simulink model "ASEComTestB"  (R2025a)
settings: Solver=ode4  StartTime=0.0  StopTime=inf  FixedStep=0.01  RelTol=1e-3
libraries: simulink x13, ASEToolBox x4
settings Model: Creator=admin  LastModifiedBy=zqhkd
settings DataIOCC: SaveFinalState=on  SaveOutput=off  InspectSignalLogs=on  SaveTime=off
settings OptimizationCC: EnhancedBackFolding=on  PassReuseOutputArgsAs=Individual arguments  ZeroExternalMemoryAtStartup=off  ZeroInternalMemoryAtStartup=off  OptimizeBlockOrder=speed  DifferentSizesBufferReuse=on  OptimizationCustomize=off  EfficientTunableParamExpr=on
settings DebuggingCC: ParameterTunabilityLossMsg=error
settings HardwareCC: ProdBitPerLong=64.0  ProdHWDeviceType=Intel->x86-64 (Linux 64)
settings SFSimCC: MATLABDynamicMemAlloc=off
settings RTWCC: SystemTargetFile=ert.tlc  TemplateMakefile=ert_default_tmf  RetainRTWFile=on  Toolchain=LCC-win64 v2.4.1 | gmake (64-bit Windows)  GPUComputeCapability=3.5  Description=Embedded Coder
settings CodeAppCC: ForceParamTrailComments=on  IgnoreCustomStorageClasses=off  OperatorAnnotations=on  SimulinkDataObjDesc=on  SFDataObjDesc=on  InsertBlockDesc=on
settings ERTTargetCC: ExtModeTransport=0.0  ExtModeStaticAlloc=off  ExtModeMexFile=ext_comm  ExtModeIntrfLevel=Level1  InlinedParameterPlacement=Hierarchical  RTWCAPISignals=on  RTWCAPIParams=on  RTWCAPIStates=on  RTWCAPIRootIO=on  ERTCustomFileTemplate=example_file_process.tlc  DynamicArrayContainerType=coder::array  TargetLangStandard=C99 (ISO)  SupportContinuousTime=on

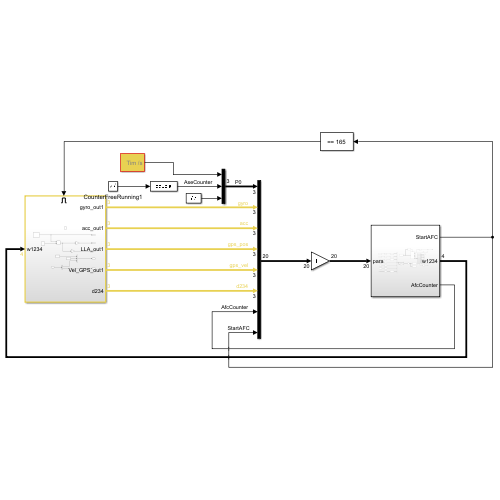
[thumbnail: Simulink's stored preview of the top-level diagram]
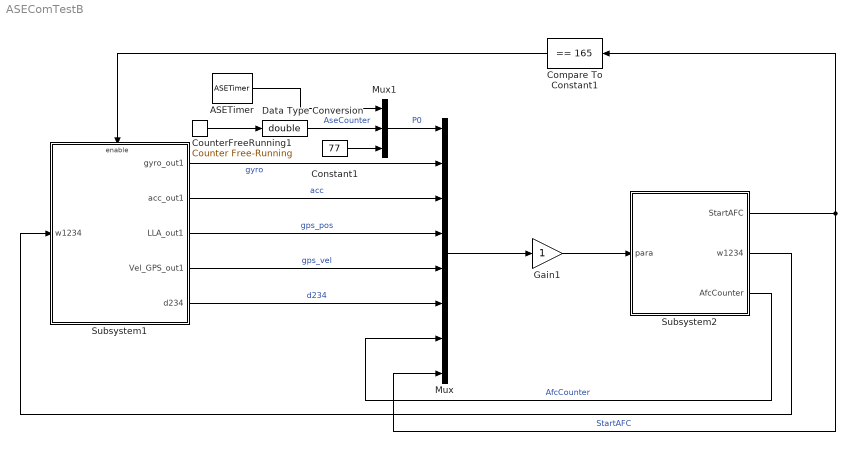
== system ASEComTestB ==
  ASETimer : ASEToolBox/SIMSystemModule/ASETimer  Priority=0  g_sampleTime=0.02
      settings: SourceProductName=ASEToolBox
  Compare To Constant1 : simulink/Logic and Bit Operations/Compare To Constant  relop===  const=165  OutDataTypeStr=boolean
  Constant1 : Constant  Value=77
  CounterFreeRunning1 : simulink/Sources/Counter Free-Running  NumBits=32  tsamp=-1
  Data Type Conversion : DataTypeConversion  OutDataTypeStr=double  SaturateOnIntegerOverflow=off  RndMeth=Floor
  Gain1 : Gain
  Mux : Mux  Inputs=8
  Mux1 : Mux  Inputs=3
  Subsystem1 : Subsystem
  Subsystem2 : Subsystem  Priority=5
  wires:
  Mux/1 -> Gain1/1
  Subsystem2/1(StartAFC) -> Mux/8, Compare To Constant1/1  "StartAFC"
  Gain1/1 -> Subsystem2/1(para)
  Compare To Constant1/1 -> Subsystem1/Enable
  Subsystem1/1(gyro_out1) -> Mux/2  "gyro"
  Subsystem1/2(acc_out1) -> Mux/3  "acc"
  Subsystem1/4(Vel_GPS_out1) -> Mux/5  "gps_vel"
  Subsystem1/5(d234) -> Mux/6  "d234"
  Subsystem2/3(AfcCounter) -> Mux/7  "AfcCounter"
  Subsystem2/2(w1234) -> Subsystem1/1(w1234)
  CounterFreeRunning1/1 -> Data Type Conversion/1
  Mux1/1 -> Mux/1  "P0"
  Subsystem1/3(LLA_out1) -> Mux/4  "gps_pos"
  ASETimer/1 -> Mux1/1
  Data Type Conversion/1 -> Mux1/2  "AseCounter"
  Constant1/1 -> Mux1/3

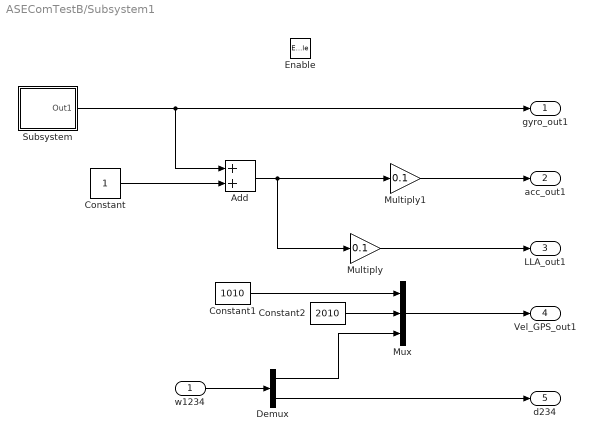
== system ASEComTestB/Subsystem1 ==
  w1234 : Inport
  Enable : EnablePort
  Add : Sum
  Constant : Constant
  Constant1 : Constant  Value=1010
  Constant2 : Constant  Value=2010
  Demux : Demux  Outputs=[1,3]
  Multiply : Gain  Gain=0.1
  Multiply1 : Gain  Gain=0.1
  Mux : Mux  Inputs=3
  Subsystem : Subsystem
  gyro_out1 : Outport
  acc_out1 : Outport  Port=2
  LLA_out1 : Outport  Port=3
  Vel_GPS_out1 : Outport  Port=4
  d234 : Outport  Port=5
  wires:
  w1234/1 -> Demux/1
  Subsystem/1(Out1) -> Add/1, gyro_out1/1
  Add/1 -> Multiply/1, Multiply1/1
  Constant/1 -> Add/2
  Multiply/1 -> LLA_out1/1
  Constant1/1 -> Mux/1
  Demux/1 -> Mux/3
  Mux/1 -> Vel_GPS_out1/1
  Demux/2 -> d234/1
  Multiply1/1 -> acc_out1/1
  Constant2/1 -> Mux/2

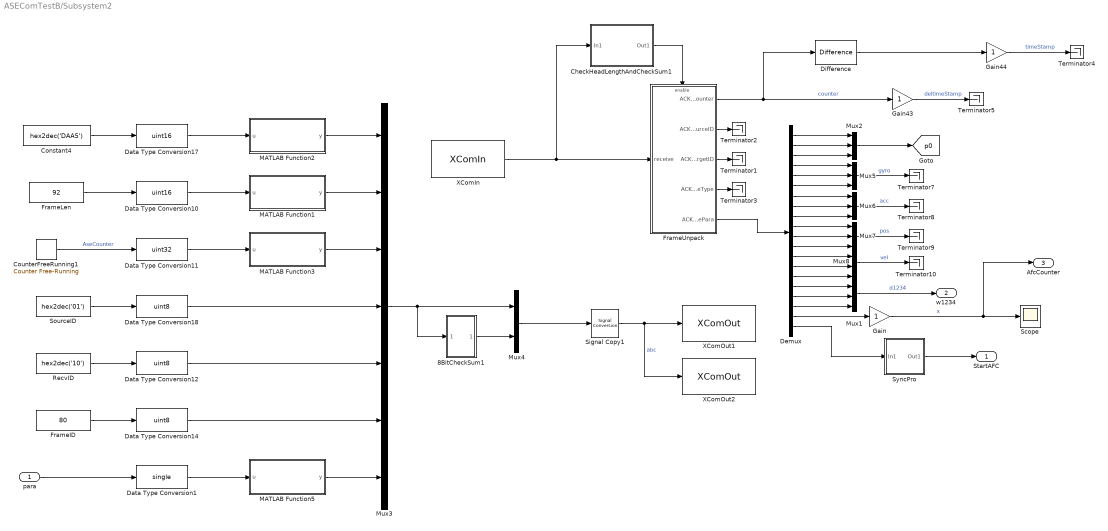
== system ASEComTestB/Subsystem2 ==
  para : Inport  PortDimensions=20
  8BitCheckSum1 : Subsystem
  CheckHeadLengthAndCheckSum1 : Subsystem
  Constant4 : Constant  Value=hex2dec('DAA5')
  CounterFreeRunning1 : simulink/Sources/Counter Free-Running  NumBits=32  tsamp=-1
  Data Type Conversion1 : DataTypeConversion  OutDataTypeStr=single  SaturateOnIntegerOverflow=off  RndMeth=Floor
  Data Type Conversion10 : DataTypeConversion  OutDataTypeStr=uint16  SaturateOnIntegerOverflow=off  RndMeth=Floor
  Data Type Conversion11 : DataTypeConversion  OutDataTypeStr=uint32  SaturateOnIntegerOverflow=off  RndMeth=Floor
  Data Type Conversion12 : DataTypeConversion  OutDataTypeStr=uint8  SaturateOnIntegerOverflow=off  RndMeth=Floor
  Data Type Conversion14 : DataTypeConversion  OutDataTypeStr=uint8  SaturateOnIntegerOverflow=off  RndMeth=Floor
  Data Type Conversion17 : DataTypeConversion  OutDataTypeStr=uint16  SaturateOnIntegerOverflow=off  RndMeth=Floor
  Data Type Conversion18 : DataTypeConversion  OutDataTypeStr=uint8  SaturateOnIntegerOverflow=off  RndMeth=Floor
  Demux : Demux  Outputs=20
  Difference : simulink/Discrete/Difference  ICPrevInput=0.0  OutMin=[]  OutMax=[]  OutDataType=fixdt(1, 16)  OutScaling=2^-10  DoSatur=off
  FrameID : Constant  Value=80
  FrameLen : Constant  Value=92
  FrameUnpack : Subsystem
  Gain : Gain
  Gain43 : Gain  OutDataTypeStr=Inherit: Same as input
  Gain44 : Gain  OutDataTypeStr=Inherit: Same as input
  MATLAB Function1 : MATLAB Function  TreatAsAtomicUnit=on
  MATLAB Function2 : MATLAB Function  TreatAsAtomicUnit=on
  MATLAB Function3 : MATLAB Function  TreatAsAtomicUnit=on
  MATLAB Function5 : MATLAB Function  TreatAsAtomicUnit=on
  Mux1 : Mux
  Mux{2,5..7} (4 alike) : Mux  Inputs=3
  Mux3 : Mux  Inputs=7
  Mux4 : Mux  Inputs=2
  Mux8 : Mux  Inputs=2
  RecvID : Constant  Value=hex2dec('10')
  Scope : Scope
  Signal Copy1 : SignalConversion  OverrideOpt=on
  SourceID : Constant  Value=hex2dec('01')
  SyncPro : Subsystem
  Terminator{1..5,7..10} (9 alike) : Terminator
  XComIn : ASEToolBox/COMModule/XComIn  g_serial_select=ttyS1  g_baudrate=460800  g_parity=None  g_databit=8  g_stopbit=0  g_data_size=92  g_sample_time=-1
      settings: SourceProductName=ASEToolBox
  XComOut1 : ASEToolBox/COMModule/XComOut  g_serial_select=ttyS1  g_baudrate=460800  g_parity=None  g_databit=8  g_stopbit=1  g_sample_time=-1
      settings: SourceProductName=ASEToolBox
  XComOut2 : ASEToolBox/COMModule/XComOut  g_serial_select=ttyS0  g_baudrate=460800  g_parity=None  g_databit=8  g_stopbit=1  g_sample_time=-1
      settings: SourceProductName=ASEToolBox
  StartAFC : Outport
  w1234 : Outport  Port=2
  AfcCounter : Outport  Port=3
  tag scope: p0=global
  wires:
  MATLAB Function5/1(y) -> Mux3/7
  Data Type Conversion12/1 -> Mux3/5
  Data Type Conversion18/1 -> Mux3/4
  para/1 -> Data Type Conversion1/1
  SourceID/1 -> Data Type Conversion18/1
  Data Type Conversion14/1 -> Mux3/6
  Mux3/1 -> 8BitCheckSum1/1(In1), Mux4/1
  Data Type Conversion11/1 -> MATLAB Function3/1(u)
  MATLAB Function3/1(y) -> Mux3/3
  Data Type Conversion1/1 -> MATLAB Function5/1(u)
  FrameLen/1 -> Data Type Conversion10/1
  FrameID/1 -> Data Type Conversion14/1
  Data Type Conversion10/1 -> MATLAB Function1/1(u)
  CounterFreeRunning1/1 -> Data Type Conversion11/1  "AseCounter"
  Data Type Conversion17/1 -> MATLAB Function2/1(u)
  Constant4/1 -> Data Type Conversion17/1
  8BitCheckSum1/1(Out1) -> Mux4/2
  MATLAB Function1/1(y) -> Mux3/2
  MATLAB Function2/1(y) -> Mux3/1
  Mux4/1 -> Signal Copy1/1
  Signal Copy1/1 -> XComOut2/1, XComOut1/1  "abc"
  Difference/1 -> Gain44/1
  FrameUnpack/3(ACKTargetID) -> Terminator1/1
  FrameUnpack/2(ACKSourceID) -> Terminator2/1
  CheckHeadLengthAndCheckSum1/1(Out1) -> FrameUnpack/Enable
  FrameUnpack/4(ACKFrameType) -> Terminator3/1
  Mux1/1 -> w1234/1  "d1234"
  FrameUnpack/1(ACKFrameCounter) -> Difference/1, Gain43/1  "counter"
  Mux2/1 -> [p0]
  FrameUnpack/5(ACKFramePara) -> Demux/1
  XComIn/1 -> FrameUnpack/1(receive), CheckHeadLengthAndCheckSum1/1(In1)
  Gain44/1 -> Terminator4/1  "timeStamp"
  Gain43/1 -> Terminator5/1  "deltimeStamp"
  RecvID/1 -> Data Type Conversion12/1
  Mux5/1 -> Terminator7/1  "gyro"
  Mux6/1 -> Terminator8/1  "acc"
  Mux7/1 -> Terminator9/1  "pos"
  Mux8/1 -> Terminator10/1  "vel"
  Gain/1 -> AfcCounter/1, Scope/1  "x"
  SyncPro/1(Out1) -> StartAFC/1
  Demux/1 -> Mux2/1
  Demux/2 -> Mux2/2
  Demux/4 -> Mux5/1
  Demux/3 -> Mux2/3
  Demux/5 -> Mux5/2
  Demux/6 -> Mux5/3
  Demux/7 -> Mux6/1
  Demux/8 -> Mux6/2
  Demux/9 -> Mux6/3
  Demux/10 -> Mux7/1
  Demux/11 -> Mux7/2
  Demux/12 -> Mux7/3
  Demux/13 -> Mux8/1
  Demux/14 -> Mux8/2
  Demux/15 -> Mux1/1
  Demux/16 -> Mux1/2
  Demux/17 -> Mux1/3
  Demux/18 -> Mux1/4
  Demux/19 -> Gain/1
  Demux/20 -> SyncPro/1(In1)

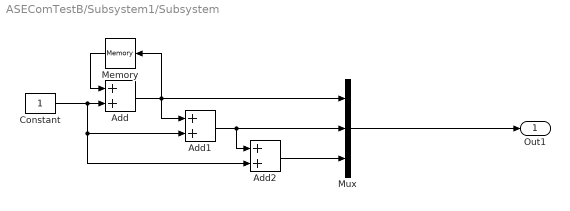
== system ASEComTestB/Subsystem1/Subsystem ==
  Add : Sum
  Add1 : Sum
  Add2 : Sum
  Constant : Constant
  Memory : Memory
  Mux : Mux  Inputs=3
  Out1 : Outport
  wires:
  Add2/1 -> Mux/3
  Constant/1 -> Add2/2, Add1/2, Add/2
  Memory/1 -> Add/1
  Add1/1 -> Add2/1, Mux/2
  Add/1 -> Memory/1, Mux/1, Add1/1
  Mux/1 -> Out1/1

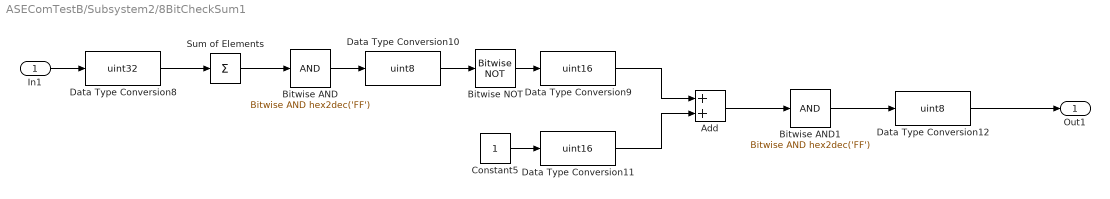
== system ASEComTestB/Subsystem2/8BitCheckSum1 ==
  In1 : Inport
  Add : Sum
  Bitwise AND : simulink/Logic and Bit Operations/Bitwise Operator  logicop=AND  UseBitMask=on  BitMask=hex2dec('FF')  BitMaskRealWorld=Stored Integer
      settings: LibrarySourceBlock=|
      | simulink/Quick Insert/Logic and Bit
      | Operations/Bitwise AND
  Bitwise AND1 : simulink/Logic and Bit Operations/Bitwise Operator  logicop=AND  UseBitMask=on  BitMask=hex2dec('FF')  BitMaskRealWorld=Stored Integer
      settings: LibrarySourceBlock=|
      | simulink/Quick Insert/Logic and Bit
      | Operations/Bitwise AND
  Bitwise NOT : simulink/Logic and Bit Operations/Bitwise Operator  logicop=NOT  UseBitMask=off  BitMask=bin2dec('11011001')  BitMaskRealWorld=Stored Integer
      settings: LibrarySourceBlock=|
      | simulink/Quick Insert/Logic and Bit
      | Operations/Bitwise NOT
  Constant5 : Constant
  Data Type Conversion10 : DataTypeConversion  OutDataTypeStr=uint8  SaturateOnIntegerOverflow=off  RndMeth=Floor
  Data Type Conversion11 : DataTypeConversion  OutDataTypeStr=uint16  SaturateOnIntegerOverflow=off  RndMeth=Floor
  Data Type Conversion12 : DataTypeConversion  OutDataTypeStr=uint8  SaturateOnIntegerOverflow=off  RndMeth=Floor
  Data Type Conversion8 : DataTypeConversion  OutDataTypeStr=uint32  SaturateOnIntegerOverflow=off  RndMeth=Floor
  Data Type Conversion9 : DataTypeConversion  OutDataTypeStr=uint16  SaturateOnIntegerOverflow=off  RndMeth=Floor
  Sum of Elements : Sum  Inputs=+
  Out1 : Outport
  wires:
  Bitwise NOT/1 -> Data Type Conversion9/1
  Constant5/1 -> Data Type Conversion11/1
  Sum of Elements/1 -> Bitwise AND/1
  Bitwise AND/1 -> Data Type Conversion10/1
  Add/1 -> Bitwise AND1/1
  Data Type Conversion9/1 -> Add/1
  Data Type Conversion11/1 -> Add/2
  Data Type Conversion8/1 -> Sum of Elements/1
  Data Type Conversion10/1 -> Bitwise NOT/1
  In1/1 -> Data Type Conversion8/1
  Data Type Conversion12/1 -> Out1/1
  Bitwise AND1/1 -> Data Type Conversion12/1

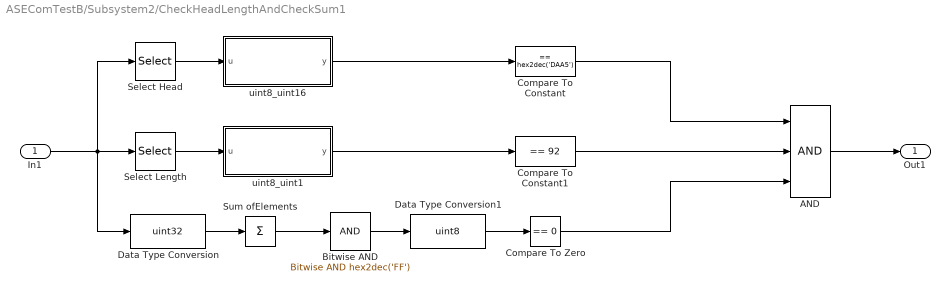
== system ASEComTestB/Subsystem2/CheckHeadLengthAndCheckSum1 ==
  In1 : Inport
  AND : Logic  Inputs=3  IconShape=distinctive  AllPortsSameDT=off  OutDataTypeStr=boolean
  Bitwise AND : simulink/Logic and Bit Operations/Bitwise Operator  logicop=AND  UseBitMask=on  BitMask=hex2dec('FF')  BitMaskRealWorld=Stored Integer
      settings: LibrarySourceBlock=|
      | simulink/Quick Insert/Logic and Bit
      | Operations/Bitwise AND
  Compare To Constant : simulink/Logic and Bit Operations/Compare To Constant  relop===  const=hex2dec('DAA5')  OutDataTypeStr=boolean
  Compare To Constant1 : simulink/Logic and Bit Operations/Compare To Constant  relop===  const=92  OutDataTypeStr=boolean
  Compare To Zero : simulink/Logic and Bit Operations/Compare To Zero  relop===  OutDataTypeStr=boolean
  Data Type Conversion : DataTypeConversion  OutDataTypeStr=uint32  SaturateOnIntegerOverflow=off  RndMeth=Floor
  Data Type Conversion1 : DataTypeConversion  OutDataTypeStr=uint8  SaturateOnIntegerOverflow=off  RndMeth=Floor
  Select Head : Selector  InputPortWidth=92  IndexOptions=Index vector (dialog)  Indices=1:2  OutputSizes=1
  Select Length : Selector  InputPortWidth=92  IndexOptions=Index vector (dialog)  Indices=3:4  OutputSizes=1
  Sum ofElements : Sum  Inputs=+
  uint8_uint1 : MATLAB Function  TreatAsAtomicUnit=on
  uint8_uint16 : MATLAB Function  TreatAsAtomicUnit=on
  Out1 : Outport
  wires:
  Sum ofElements/1 -> Bitwise AND/1
  Data Type Conversion1/1 -> Compare To Zero/1
  Select Length/1 -> uint8_uint1/1(u)
  Compare To Constant/1 -> AND/1
  AND/1 -> Out1/1
  Data Type Conversion/1 -> Sum ofElements/1
  uint8_uint16/1(y) -> Compare To Constant/1
  Compare To Zero/1 -> AND/3
  Bitwise AND/1 -> Data Type Conversion1/1
  Select Head/1 -> uint8_uint16/1(u)
  Compare To Constant1/1 -> AND/2
  uint8_uint1/1(y) -> Compare To Constant1/1
  In1/1 -> Data Type Conversion/1, Select Length/1, Select Head/1

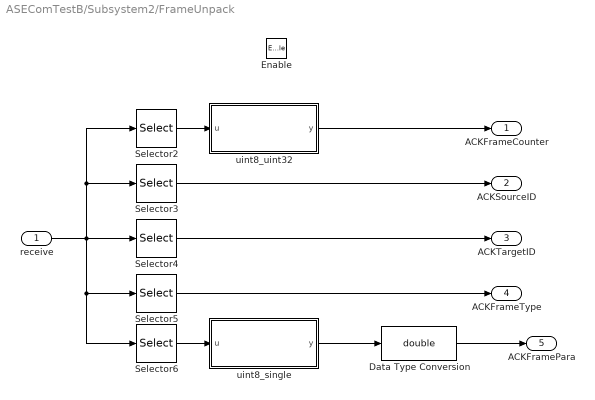
== system ASEComTestB/Subsystem2/FrameUnpack ==
  receive : Inport
  Enable : EnablePort
  Data Type Conversion : DataTypeConversion  OutDataTypeStr=double  SaturateOnIntegerOverflow=off  RndMeth=Floor
  Selector2 : Selector  InputPortWidth=92  IndexOptions=Index vector (dialog)  Indices=5:8  OutputSizes=1
  Selector3 : Selector  InputPortWidth=92  IndexOptions=Index vector (dialog)  Indices=9  OutputSizes=1
  Selector4 : Selector  InputPortWidth=92  IndexOptions=Index vector (dialog)  Indices=10  OutputSizes=1
  Selector5 : Selector  InputPortWidth=92  IndexOptions=Index vector (dialog)  Indices=11  OutputSizes=1
  Selector6 : Selector  InputPortWidth=92  IndexOptions=Index vector (dialog)  Indices=12:91  OutputSizes=1
  uint8_single : MATLAB Function  TreatAsAtomicUnit=on
  uint8_uint32 : MATLAB Function  TreatAsAtomicUnit=on
  ACKFrameCounter : Outport
  ACKSourceID : Outport  Port=2
  ACKTargetID : Outport  Port=3
  ACKFrameType : Outport  Port=4
  ACKFramePara : Outport  Port=5
  wires:
  Selector2/1 -> uint8_uint32/1(u)
  Selector3/1 -> ACKSourceID/1
  Selector4/1 -> ACKTargetID/1
  Selector5/1 -> ACKFrameType/1
  Selector6/1 -> uint8_single/1(u)
  Data Type Conversion/1 -> ACKFramePara/1
  uint8_uint32/1(y) -> ACKFrameCounter/1
  receive/1 -> Selector6/1, Selector5/1, Selector4/1, Selector3/1, Selector2/1
  uint8_single/1(y) -> Data Type Conversion/1

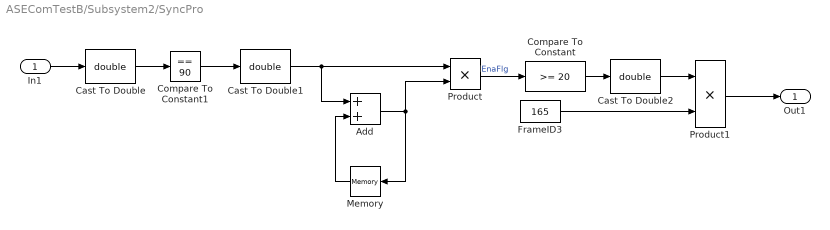
== system ASEComTestB/Subsystem2/SyncPro ==
  In1 : Inport
  Add : Sum
  Cast To Double : DataTypeConversion  OutDataTypeStr=double  SaturateOnIntegerOverflow=off  RndMeth=Floor
  Cast To Double1 : DataTypeConversion  OutDataTypeStr=double  SaturateOnIntegerOverflow=off  RndMeth=Floor
  Cast To Double2 : DataTypeConversion  OutDataTypeStr=double  SaturateOnIntegerOverflow=off  RndMeth=Floor
  Compare To Constant : simulink/Logic and Bit Operations/Compare To Constant  relop=>=  const=20  OutDataTypeStr=boolean
  Compare To Constant1 : simulink/Logic and Bit Operations/Compare To Constant  relop===  const=90  OutDataTypeStr=boolean
  FrameID3 : Constant  Value=165
  Memory : Memory
  Product : Product
  Product1 : Product
  Out1 : Outport
  wires:
  Memory/1 -> Add/2
  Cast To Double2/1 -> Product1/1
  Compare To Constant/1 -> Cast To Double2/1
  FrameID3/1 -> Product1/2
  Product/1 -> Compare To Constant/1  "EnaFlg"
  In1/1 -> Cast To Double/1
  Cast To Double1/1 -> Product/1, Add/1
  Compare To Constant1/1 -> Cast To Double1/1
  Cast To Double/1 -> Compare To Constant1/1
  Add/1 -> Product/2, Memory/1
  Product1/1 -> Out1/1

== matlab function ASEComTestB/Subsystem2/MATLAB Function1 ==
  data: u input; y output
function y = ToUint16Bytes(u)

inputType = class(u);%

if ~isa(inputType,'uint16')
    u = uint16(u);
end

temBytes = typecast(u,'uint8');

Len = length(temBytes);

y = uint8(zeros(2,1));

if Len >= 1    
    for k=1:2
        y(k) = temBytes(k);
    end
end
end

== matlab function ASEComTestB/Subsystem2/FrameUnpack/uint8_single ==
  data: u input uint8 size=[1 80]; y output single size=20
function y  = fcn(u)

num = uint32(20);%解析后数据的个数，由10个变为20个浮点数

Len = uint32(length(u));%原始uint8类型数据长度

y = single(zeros(num,1));%初始化

if ((num*4)==Len)    
    for k=1:num
        y(k) = typecast(u(k*4-3:k*4),'single');
    end
end
end

== matlab function ASEComTestB/Subsystem2/MATLAB Function2 ==
  data: u input; y output
function y = ToUint16Bytes(u)

inputType = class(u);%

if ~isa(inputType,'uint16')
    u = uint16(u);
end

temBytes = typecast(u,'uint8');

Len = length(temBytes);

y = uint8(zeros(2,1));

if Len >= 1    
    for k=1:2
        y(k) = temBytes(k);
    end
end
end

== matlab function ASEComTestB/Subsystem2/MATLAB Function3 ==
  data: u input; y output
function y = ToUint32Bytes(u)

inputType = class(u);%

if ~isa(inputType,'uint32')
    u = uint32(u);
end

temBytes = typecast(u,'uint8');

Len = length(temBytes);

y = uint8(zeros(4,1));

if Len >= 1    
    for k=1:4
        y(k) = temBytes(k);
    end
end
end

== matlab function ASEComTestB/Subsystem2/MATLAB Function5 ==
  data: u input size=[20 1]; y output
function y = ToSingleBytes(u)

inputType = class(u);%
num = 20;
if ~isa(inputType,'single')
    u = single(u);
end

temBytes = typecast(u,'uint8');

Len = length(temBytes);

y = uint8(zeros(4*num,1));

if Len >= 1    
    for k=1:4*num
        y(k) = temBytes(k);
    end
end
end

== matlab function ASEComTestB/Subsystem2/CheckHeadLengthAndCheckSum1/uint8_uint1 ==
  data: u input uint8; y output uint16 size=1
function y = fcn(u)

y = uint16(typecast(u,'uint16'));

== matlab function ASEComTestB/Subsystem2/CheckHeadLengthAndCheckSum1/uint8_uint16 ==
  data: u input uint8; y output uint16 size=1
function y = fcn(u)

y = uint16(typecast(u,'uint16'));

== matlab function ASEComTestB/Subsystem2/FrameUnpack/uint8_uint32 ==
  data: u input uint8 size=[1 4]; y output uint32 size=1
function y = fcn(u)

y = uint32(typecast(u,'uint32'));
